simulink model "quad_six"  (R2025b)
settings: Solver=ode8  StartTime=0.0  StopTime=10.0  FixedStep=0.01  RelTol=1e-3
settings Model: Creator=MehrSystem  LastModifiedBy=MehrSystem

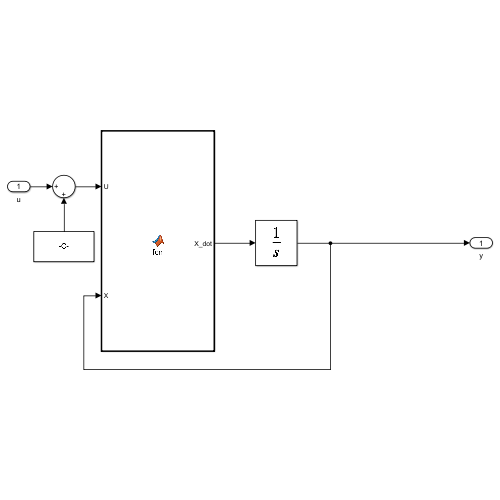
[thumbnail: Simulink's stored preview of the top-level diagram]
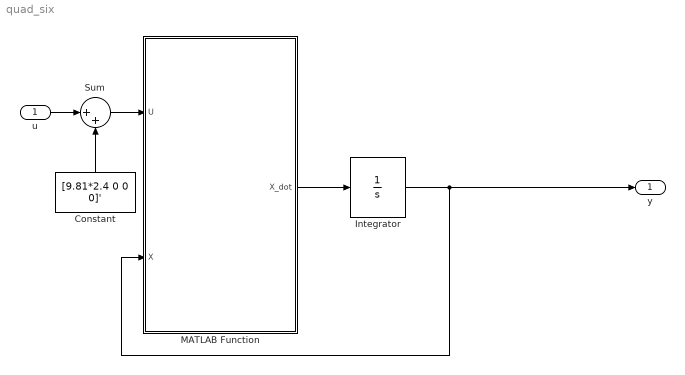
== system quad_six ==
  u : Inport
  Constant : Constant  Value=[9.81*2.4 0 0 0]'
  Integrator : Integrator  InitialCondition=[0 0 0 0 0 0 0 0 0 0 0 0]'
  MATLAB Function : MATLAB Function  TreatAsAtomicUnit=on
  Sum : Sum  Inputs=|++
  y : Outport
  wires:
  MATLAB Function/1(X_dot) -> Integrator/1
  Constant/1 -> Sum/2
  u/1 -> Sum/1
  Integrator/1 -> y/1, MATLAB Function/2(X)
  Sum/1 -> MATLAB Function/1(U)

== matlab function quad_six/MATLAB Function ==
  data: U input; X_dot output; X input
function X_dot = fcn(U, X)
x = X(1);
y = X(2);
z = X(3);
phi = X(4);
theta = X(5);
psi = X(6);
u = X(7);
v = X(8);
w = X(9);
p = X(10);
q = X(11);
r = X(12);
U1 = U(1);
U2 = U(2);
U3 = U(3);
U4 = U(4);
g = 9.81;
m = 2.4; %(Kg)
Ix = 0.04; %(Kg m^2)
Iy = 0.04; %(Kg m^2)
Iz = 0.08; %(Kg m^2)
x_dot = u * (cos(psi)*cos(theta)) + v * (cos(psi)*sin(theta)*sin(phi) - cos(phi)*sin(psi)) + ...
        w * (cos(psi)*sin(theta)*cos(phi) + sin(psi)*sin(phi));
y_dot = u * (cos(theta)*sin(psi)) + v * (sin(psi)*sin(theta)*sin(phi) + cos(phi)*cos(psi)) + ...
        w * (sin(psi)*sin(theta)*cos(phi) - cos(psi)*sin(phi));
z_dot = u * (-sin(theta)) + v * (cos(theta)*sin(phi)) + w * (cos(theta)*cos(phi));
phi_dot = p + q * sin(phi)*tan(theta) + r * cos(phi)*tan(theta);
theta_dot = q * cos(phi) - r * sin(phi);
psi_dot = q * sin(phi)/cos(theta) + r * cos(phi)/cos(theta);
u_dot = g*sin(theta);
v_dot = -g*cos(theta)*sin(phi);
w_dot = -g*cos(theta)*cos(phi) + U1/m;
p_dot = U2/Ix + q*r*(Iy-Iz)/Ix;
q_dot = U3/Iy + r*p*(Iz-Ix)/Ix;
r_dot = U4/Iz + p*q*(Ix-Iy)/Iz;
X_dot = [x_dot y_dot z_dot phi_dot theta_dot psi_dot u_dot v_dot w_dot p_dot q_dot r_dot]';
